simulink subsystem "Subsys_Conv_Ctrl_meas_Protection"  (R2022b)
settings: Solver=VariableStepAuto  StartTime=0.0  StopTime=10.0  RelTol=1e-3
model mask{prot_variant=1, f_n=50, meas_signals=0, v_n_dc=sqrt(6), v_dc_max=1.2*sqrt(6), v_ac_max=1.1, t_ac_max=0.1, v_ac_maxmax=1.25, t_ac_maxmax=0.1, v_ac_min=0.8, t_ac_min=3, v_ac_minmin=0.45, t_ac_minmin=0.3, f_ac_max=51.5, t_f_ac_max=0.1, f_ac_maxmax=52.5, t_f_ac_maxmax=10, f_ac_min=47.5, t_f_ac_min=0.1, i_ac_max=1.25, T_s=1e-4}
  mask prompts: prot_variant "Protection Variant (1 = hardware protection, 2 = tDMSquared warnings only, 3 = deactivated, 4 = VDE AR)"; f_n "Nominal frequency"; meas_signals "Measurement signals (0 = all signals (tDMSquared simulation), 1 = reduced (imperix hardware))"; v_n_dc "Nominal DC-link voltage [pu]"; v_dc_max "Maximum DC-link voltage [pu]"; v_ac_max "Maximum AC voltage amplitude [pu]"; t_ac_max "Maximum AC voltage amplitude timing"; v_ac_maxmax "Upper Maximum AC voltage amplitude [pu]"; t_ac_maxmax "Upper Maximum AC voltage amplitude timing"; v_ac_min "Upper Minimum AC voltage amplitude [pu]"; t_ac_min "Upper Minimum AC voltage amplitude timing"; v_ac_minmin "Lower Minimum AC voltage amplitude [pu]"; t_ac_minmin "Lower Minimum AC voltage amplitude timing"; f_ac_max "Maximum AC voltage frequency [Hz]"; t_f_ac_max "Maximum AC voltage frequency timing"; f_ac_maxmax "Upper Maximum AC voltage frequency [Hz]"; t_f_ac_maxmax "Upper Maximum AC voltage frequency timing"; f_ac_min "Minimum AC voltage frequency [Hz]"; t_f_ac_min "Minimum AC voltage frequencytiming"; i_ac_max "Maximum AC current amplitude [pu]"; T_s "Sample Time [s]"
undefined symbols (not defined in the file): DiscIntNeverNeededParam
libraries: simulink x63, spsRMSLib x1
settings Model: DefaultTestHarness=Subsys_Conv_Ctrl_meas_Protection_Harness1  Creator=winkens  LastModifiedBy=m.stroot
settings SolverCC: AlgebraicLoopSolver=TrustRegion
settings DebuggingCC: UnconnectedInputMsg=warning  UnconnectedOutputMsg=warning  UnconnectedLineMsg=warning  SFMachineParentedDataDiag=warning
settings ModelReferenceCC: EnableRefExpFcnMdlSchedulingChecks=on
settings RTWCC: DLArmComputeVersion=19.05

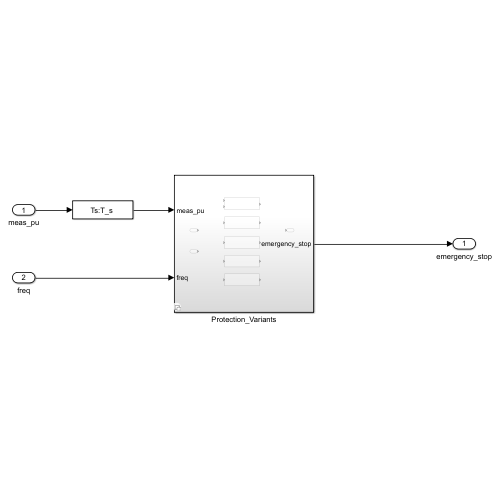
[thumbnail: Simulink's stored preview of the top-level diagram]
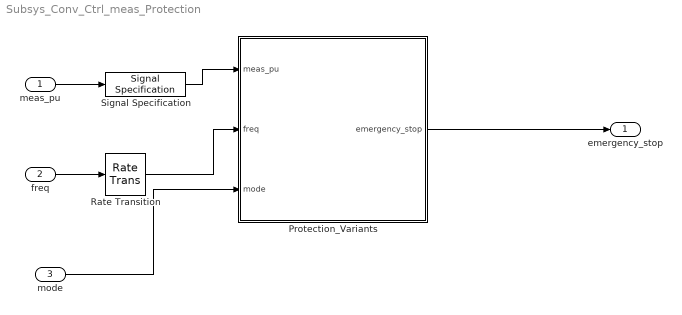
== system Subsys_Conv_Ctrl_meas_Protection ==
  meas_pu : Inport
  freq : Inport  Port=2
  mode : Inport  Port=3
  Protection_Variants : Subsystem  Variant=on
  Rate Transition : RateTransition  OutPortSampleTime=T_s
  Signal Specification : SignalSpecification  SampleTime=T_s
  emergency_stop : Outport  OutDataTypeStr=boolean
  wires:
  mode/1 -> Protection_Variants/3(mode)
  freq/1 -> Rate Transition/1
  Signal Specification/1 -> Protection_Variants/1(meas_pu)
  meas_pu/1 -> Signal Specification/1
  Protection_Variants/1(emergency_stop) -> emergency_stop/1
  Rate Transition/1 -> Protection_Variants/2(freq)

== system Subsys_Conv_Ctrl_meas_Protection/Protection_Variants ==
  meas_pu : Inport
  freq : Inport  Port=2
  mode : Inport  Port=3
  Hardware_Protection : Subsystem  VariantControl=(prot_variant == 1) && (meas_signals == 0)
  Hardware_Protection_imperix : Subsystem  VariantControl=(prot_variant == 1) && (meas_signals == 1)
  No_Protection : Subsystem  VariantControl=prot_variant == 3
  VDE_AR : Subsystem  VariantControl=(prot_variant == 4)
  tDMSquared_Warnings : Subsystem  VariantControl=prot_variant == 2
  emergency_stop : Outport

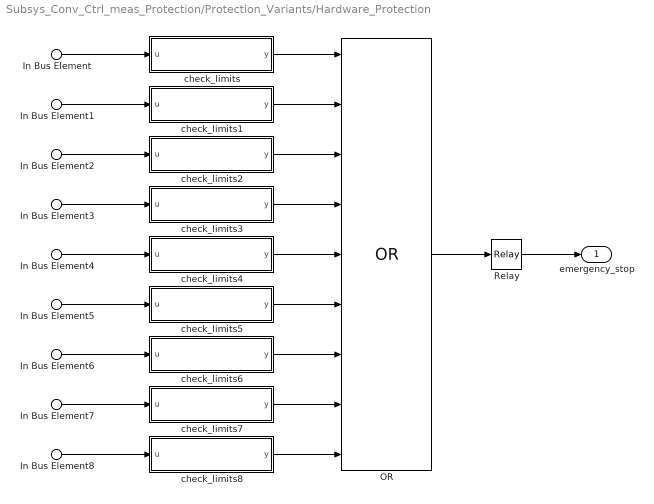
== system Subsys_Conv_Ctrl_meas_Protection/Protection_Variants/Hardware_Protection ==
  In Bus Element : Inport  PortName=meas_pu  Element=v_dc
  In Bus Element1 : Inport  PortName=meas_pu  Element=v_dc_up
  In Bus Element2 : Inport  PortName=meas_pu  Element=v_dc_low
  In Bus Element3 : Inport  PortName=meas_pu  Element=v_cap_abc
  In Bus Element4 : Inport  PortName=meas_pu  Element=v_breaker_abc
  In Bus Element5 : Inport  PortName=meas_pu  Element=v_grid_abc
  In Bus Element6 : Inport  PortName=meas_pu  Element=i_conv_abc
  In Bus Element7 : Inport  PortName=meas_pu  Element=i_filter_grid_abc
  In Bus Element8 : Inport  PortName=meas_pu  Element=i_grid_abc
  OR : Logic  Operator=OR  Inputs=9  AllPortsSameDT=off  OutDataTypeStr='double'
  Relay : Relay  OnSwitchValue=0.5  OffSwitchValue=-0.5  OutDataTypeStr=boolean
  check_limits : Subsystem
  check_limits1 : Subsystem
  check_limits2 : Subsystem
  check_limits3 : Subsystem
  check_limits4 : Subsystem
  check_limits5 : Subsystem
  check_limits6 : Subsystem
  check_limits7 : Subsystem
  check_limits8 : Subsystem
  emergency_stop : Outport
  wires:
  Relay/1 -> emergency_stop/1
  OR/1 -> Relay/1
  check_limits8/1(y) -> OR/9
  check_limits7/1(y) -> OR/8
  check_limits6/1(y) -> OR/7
  check_limits5/1(y) -> OR/6
  check_limits4/1(y) -> OR/5
  check_limits3/1(y) -> OR/4
  check_limits2/1(y) -> OR/3
  check_limits1/1(y) -> OR/2
  check_limits/1(y) -> OR/1
  In Bus Element8/1 -> check_limits8/1(u)
  In Bus Element7/1 -> check_limits7/1(u)
  In Bus Element6/1 -> check_limits6/1(u)
  In Bus Element4/1 -> check_limits4/1(u)
  In Bus Element5/1 -> check_limits5/1(u)
  In Bus Element3/1 -> check_limits3/1(u)
  In Bus Element2/1 -> check_limits2/1(u)
  In Bus Element1/1 -> check_limits1/1(u)
  In Bus Element/1 -> check_limits/1(u)

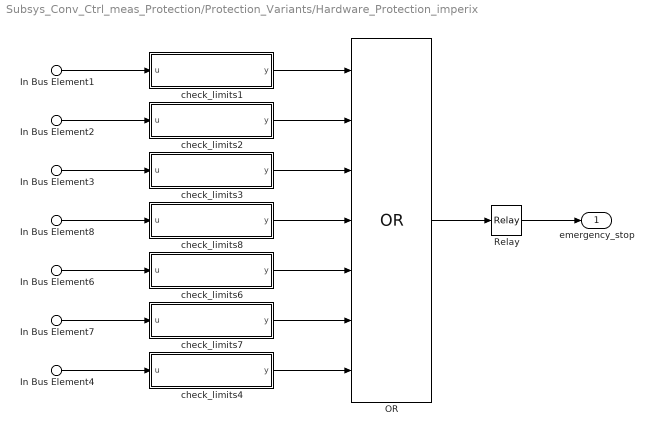
== system Subsys_Conv_Ctrl_meas_Protection/Protection_Variants/Hardware_Protection_imperix ==
  In Bus Element1 : Inport  PortName=meas_pu  Element=v_dc_up
  In Bus Element2 : Inport  PortName=meas_pu  Element=v_dc_low
  In Bus Element3 : Inport  PortName=meas_pu  Element=v_cap_ab-bc-ca
  In Bus Element6 : Inport  PortName=meas_pu  Element=i_conv2_abc
  In Bus Element7 : Inport  PortName=meas_pu  Element=i_filter_grid_abc
  In Bus Element8 : Inport  PortName=meas_pu  Element=i_conv1_abc
  In Bus Element4 : Inport  PortName=meas_pu  Element=i_filter_grid_n
  OR : Logic  Operator=OR  Inputs=7  AllPortsSameDT=off  OutDataTypeStr='double'
  Relay : Relay  OnSwitchValue=0.5  OffSwitchValue=-0.5  OutDataTypeStr=boolean
  check_limits1 : Subsystem
  check_limits2 : Subsystem
  check_limits3 : Subsystem
  check_limits4 : Subsystem
  check_limits6 : Subsystem
  check_limits7 : Subsystem
  check_limits8 : Subsystem
  emergency_stop : Outport
  wires:
  In Bus Element4/1 -> check_limits4/1(u)
  check_limits4/1(y) -> OR/7
  Relay/1 -> emergency_stop/1
  OR/1 -> Relay/1
  check_limits8/1(y) -> OR/4
  check_limits7/1(y) -> OR/6
  check_limits6/1(y) -> OR/5
  check_limits3/1(y) -> OR/3
  check_limits2/1(y) -> OR/2
  check_limits1/1(y) -> OR/1
  In Bus Element8/1 -> check_limits8/1(u)
  In Bus Element7/1 -> check_limits7/1(u)
  In Bus Element6/1 -> check_limits6/1(u)
  In Bus Element3/1 -> check_limits3/1(u)
  In Bus Element2/1 -> check_limits2/1(u)
  In Bus Element1/1 -> check_limits1/1(u)

== system Subsys_Conv_Ctrl_meas_Protection/Protection_Variants/No_Protection ==
  meas_pu : Inport
  Ground : Ground
  Terminator : Terminator
  emergency_stop : Outport
  wires:
  Ground/1 -> emergency_stop/1
  meas_pu/1 -> Terminator/1

== system Subsys_Conv_Ctrl_meas_Protection/Protection_Variants/VDE_AR ==
  In Bus Element1 : Inport  PortName=meas_pu  Element=v_breaker_abc
  freq : Inport  Port=2
  mode : Inport  Port=3
  Compare To Constant : simulink/Logic and Bit Operations/Compare To Constant  relop=>  const=1  OutDataTypeStr=boolean
  Subsystem : Subsystem
  emergency_stop : Outport
  wires:
  In Bus Element1/1 -> Subsystem/1(In1)
  freq/1 -> Subsystem/2(freq)
  Subsystem/1(emergency_stop) -> emergency_stop/1
  mode/1 -> Compare To Constant/1
  Compare To Constant/1 -> Subsystem/Enable

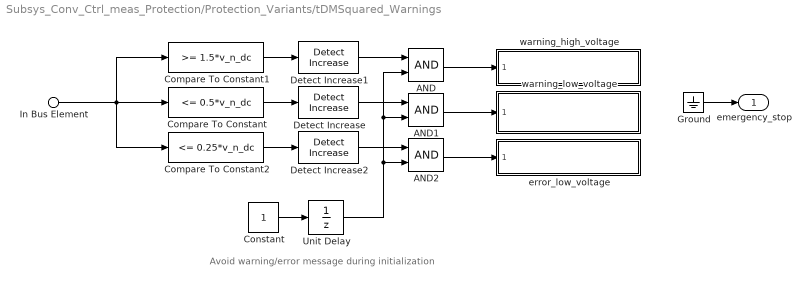
== system Subsys_Conv_Ctrl_meas_Protection/Protection_Variants/tDMSquared_Warnings ==
  note: Avoid warning/error message during initialization
  In Bus Element : Inport  PortName=meas_pu  Element=v_dc
  AND : Logic  AllPortsSameDT=off  OutDataTypeStr=boolean
  AND1 : Logic  AllPortsSameDT=off  OutDataTypeStr=boolean
  AND2 : Logic  AllPortsSameDT=off  OutDataTypeStr=boolean
  Compare To Constant : simulink/Logic and Bit Operations/Compare To Constant  relop=<=  const=0.5*v_n_dc  OutDataTypeStr=boolean
  Compare To Constant1 : simulink/Logic and Bit Operations/Compare To Constant  relop=>=  const=1.5*v_n_dc  OutDataTypeStr=boolean
  Compare To Constant2 : simulink/Logic and Bit Operations/Compare To Constant  relop=<=  const=0.25*v_n_dc  OutDataTypeStr=boolean
  Constant : Constant  OutDataTypeStr=boolean
  Detect Increase : simulink/Logic and Bit Operations/Detect Increase  vinit=0.0  OutDataTypeStr=boolean
  Detect Increase1 : simulink/Logic and Bit Operations/Detect Increase  vinit=0.0  OutDataTypeStr=boolean
  Detect Increase2 : simulink/Logic and Bit Operations/Detect Increase  vinit=0.0  OutDataTypeStr=boolean
  Ground : Ground
  Unit Delay : UnitDelay  SampleTime=T_s  HasFrameUpgradeWarning=on
  error_low_voltage : Subsystem  ReferencedSubsystem=tDMSquared_Error  messageText='DC-Link Voltage dropped below 25% of its nominal value. The simulation is terminated.'  T_s=T_s  stopSim=on
  warning_high_voltage : Subsystem  ReferencedSubsystem=tDMSquared_Warning  messageText='DC-Link Voltage increased to 150% of its nominal value. The results of the following timesteps need to be revisited.'  T_s=T_s
  warning_low_voltage : Subsystem  ReferencedSubsystem=tDMSquared_Warning  messageText='DC-Link Voltage dropped below 50% of its nominal value. The results of the following timesteps need to be revisited.'  T_s=T_s
  emergency_stop : Outport
  wires:
  Unit Delay/1 -> AND1/2, AND/2, AND2/2
  AND2/1 -> error_low_voltage/1
  AND1/1 -> warning_low_voltage/1
  AND/1 -> warning_high_voltage/1
  Constant/1 -> Unit Delay/1
  Compare To Constant/1 -> Detect Increase/1
  Compare To Constant2/1 -> Detect Increase2/1
  Detect Increase/1 -> AND1/1
  Compare To Constant1/1 -> Detect Increase1/1
  In Bus Element/1 -> Compare To Constant/1, Compare To Constant1/1, Compare To Constant2/1
  Detect Increase1/1 -> AND/1
  Detect Increase2/1 -> AND2/1
  Ground/1 -> emergency_stop/1

== system Subsys_Conv_Ctrl_meas_Protection/Protection_Variants/Hardware_Protection/check_limits ==
  u : Inport
  Compare To Constant1 : simulink/Logic and Bit Operations/Compare To Constant  relop=>=  const=v_dc_max  OutDataTypeStr=boolean
  y : Outport
  wires:
  u/1 -> Compare To Constant1/1
  Compare To Constant1/1 -> y/1

== system Subsys_Conv_Ctrl_meas_Protection/Protection_Variants/Hardware_Protection/check_limits1 ==
  u : Inport
  Compare To Constant1 : simulink/Logic and Bit Operations/Compare To Constant  relop=>=  const=0.5*v_dc_max  OutDataTypeStr=boolean
  y : Outport
  wires:
  u/1 -> Compare To Constant1/1
  Compare To Constant1/1 -> y/1

== system Subsys_Conv_Ctrl_meas_Protection/Protection_Variants/Hardware_Protection/check_limits2 ==
  u : Inport
  Compare To Constant1 : simulink/Logic and Bit Operations/Compare To Constant  relop=>=  const=0.5*v_dc_max  OutDataTypeStr=boolean
  y : Outport
  wires:
  u/1 -> Compare To Constant1/1
  Compare To Constant1/1 -> y/1

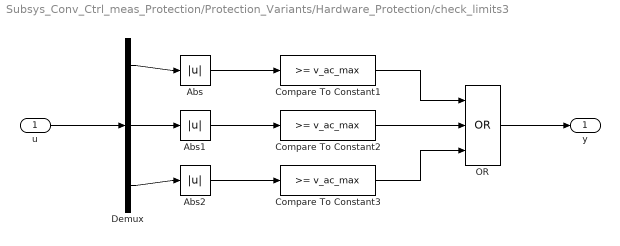
== system Subsys_Conv_Ctrl_meas_Protection/Protection_Variants/Hardware_Protection/check_limits3 ==
  u : Inport
  Abs : Abs  SaturateOnIntegerOverflow=off
  Abs1 : Abs  SaturateOnIntegerOverflow=off
  Abs2 : Abs  SaturateOnIntegerOverflow=off
  Compare To Constant1 : simulink/Logic and Bit Operations/Compare To Constant  relop=>=  const=v_ac_max  OutDataTypeStr=boolean
  Compare To Constant2 : simulink/Logic and Bit Operations/Compare To Constant  relop=>=  const=v_ac_max  OutDataTypeStr=boolean
  Compare To Constant3 : simulink/Logic and Bit Operations/Compare To Constant  relop=>=  const=v_ac_max  OutDataTypeStr=boolean
  Demux : Demux  Outputs=3
  OR : Logic  Operator=OR  Inputs=3  AllPortsSameDT=off  OutDataTypeStr=boolean
  y : Outport
  wires:
  OR/1 -> y/1
  Compare To Constant3/1 -> OR/3
  Compare To Constant1/1 -> OR/1
  Compare To Constant2/1 -> OR/2
  Abs2/1 -> Compare To Constant3/1
  Abs1/1 -> Compare To Constant2/1
  Abs/1 -> Compare To Constant1/1
  Demux/3 -> Abs2/1
  Demux/2 -> Abs1/1
  Demux/1 -> Abs/1
  u/1 -> Demux/1

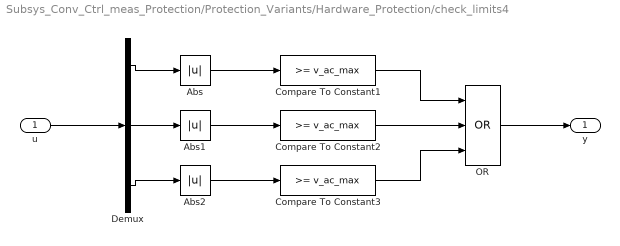
== system Subsys_Conv_Ctrl_meas_Protection/Protection_Variants/Hardware_Protection/check_limits4 ==
  u : Inport
  Abs : Abs  SaturateOnIntegerOverflow=off
  Abs1 : Abs  SaturateOnIntegerOverflow=off
  Abs2 : Abs  SaturateOnIntegerOverflow=off
  Compare To Constant1 : simulink/Logic and Bit Operations/Compare To Constant  relop=>=  const=v_ac_max  OutDataTypeStr=boolean
  Compare To Constant2 : simulink/Logic and Bit Operations/Compare To Constant  relop=>=  const=v_ac_max  OutDataTypeStr=boolean
  Compare To Constant3 : simulink/Logic and Bit Operations/Compare To Constant  relop=>=  const=v_ac_max  OutDataTypeStr=boolean
  Demux : Demux  Outputs=3
  OR : Logic  Operator=OR  Inputs=3  AllPortsSameDT=off  OutDataTypeStr=boolean
  y : Outport
  wires:
  OR/1 -> y/1
  Compare To Constant3/1 -> OR/3
  Compare To Constant1/1 -> OR/1
  Compare To Constant2/1 -> OR/2
  Abs2/1 -> Compare To Constant3/1
  Abs1/1 -> Compare To Constant2/1
  Abs/1 -> Compare To Constant1/1
  Demux/3 -> Abs2/1
  Demux/2 -> Abs1/1
  Demux/1 -> Abs/1
  u/1 -> Demux/1

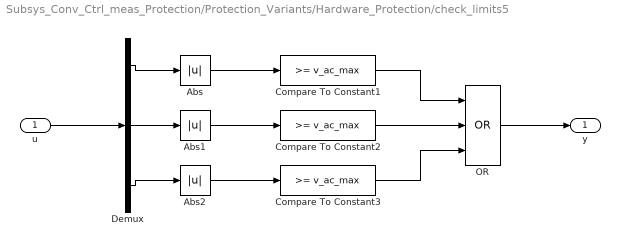
== system Subsys_Conv_Ctrl_meas_Protection/Protection_Variants/Hardware_Protection/check_limits5 ==
  u : Inport
  Abs : Abs  SaturateOnIntegerOverflow=off
  Abs1 : Abs  SaturateOnIntegerOverflow=off
  Abs2 : Abs  SaturateOnIntegerOverflow=off
  Compare To Constant1 : simulink/Logic and Bit Operations/Compare To Constant  relop=>=  const=v_ac_max  OutDataTypeStr=boolean
  Compare To Constant2 : simulink/Logic and Bit Operations/Compare To Constant  relop=>=  const=v_ac_max  OutDataTypeStr=boolean
  Compare To Constant3 : simulink/Logic and Bit Operations/Compare To Constant  relop=>=  const=v_ac_max  OutDataTypeStr=boolean
  Demux : Demux  Outputs=3
  OR : Logic  Operator=OR  Inputs=3  AllPortsSameDT=off  OutDataTypeStr=boolean
  y : Outport
  wires:
  OR/1 -> y/1
  Compare To Constant3/1 -> OR/3
  Compare To Constant1/1 -> OR/1
  Compare To Constant2/1 -> OR/2
  Abs2/1 -> Compare To Constant3/1
  Abs1/1 -> Compare To Constant2/1
  Abs/1 -> Compare To Constant1/1
  Demux/3 -> Abs2/1
  Demux/2 -> Abs1/1
  Demux/1 -> Abs/1
  u/1 -> Demux/1

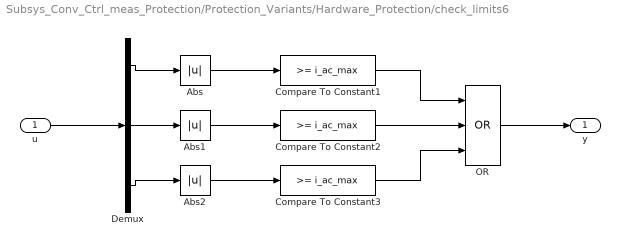
== system Subsys_Conv_Ctrl_meas_Protection/Protection_Variants/Hardware_Protection/check_limits6 ==
  u : Inport
  Abs : Abs  SaturateOnIntegerOverflow=off
  Abs1 : Abs  SaturateOnIntegerOverflow=off
  Abs2 : Abs  SaturateOnIntegerOverflow=off
  Compare To Constant1 : simulink/Logic and Bit Operations/Compare To Constant  relop=>=  const=i_ac_max  OutDataTypeStr=boolean
  Compare To Constant2 : simulink/Logic and Bit Operations/Compare To Constant  relop=>=  const=i_ac_max  OutDataTypeStr=boolean
  Compare To Constant3 : simulink/Logic and Bit Operations/Compare To Constant  relop=>=  const=i_ac_max  OutDataTypeStr=boolean
  Demux : Demux  Outputs=3
  OR : Logic  Operator=OR  Inputs=3  AllPortsSameDT=off  OutDataTypeStr=boolean
  y : Outport
  wires:
  OR/1 -> y/1
  Compare To Constant3/1 -> OR/3
  Compare To Constant1/1 -> OR/1
  Compare To Constant2/1 -> OR/2
  Abs2/1 -> Compare To Constant3/1
  Abs1/1 -> Compare To Constant2/1
  Abs/1 -> Compare To Constant1/1
  Demux/3 -> Abs2/1
  Demux/2 -> Abs1/1
  Demux/1 -> Abs/1
  u/1 -> Demux/1

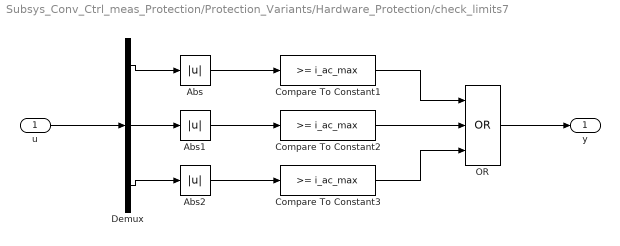
== system Subsys_Conv_Ctrl_meas_Protection/Protection_Variants/Hardware_Protection/check_limits7 ==
  u : Inport
  Abs : Abs  SaturateOnIntegerOverflow=off
  Abs1 : Abs  SaturateOnIntegerOverflow=off
  Abs2 : Abs  SaturateOnIntegerOverflow=off
  Compare To Constant1 : simulink/Logic and Bit Operations/Compare To Constant  relop=>=  const=i_ac_max  OutDataTypeStr=boolean
  Compare To Constant2 : simulink/Logic and Bit Operations/Compare To Constant  relop=>=  const=i_ac_max  OutDataTypeStr=boolean
  Compare To Constant3 : simulink/Logic and Bit Operations/Compare To Constant  relop=>=  const=i_ac_max  OutDataTypeStr=boolean
  Demux : Demux  Outputs=3
  OR : Logic  Operator=OR  Inputs=3  AllPortsSameDT=off  OutDataTypeStr=boolean
  y : Outport
  wires:
  OR/1 -> y/1
  Compare To Constant3/1 -> OR/3
  Compare To Constant1/1 -> OR/1
  Compare To Constant2/1 -> OR/2
  Abs2/1 -> Compare To Constant3/1
  Abs1/1 -> Compare To Constant2/1
  Abs/1 -> Compare To Constant1/1
  Demux/3 -> Abs2/1
  Demux/2 -> Abs1/1
  Demux/1 -> Abs/1
  u/1 -> Demux/1

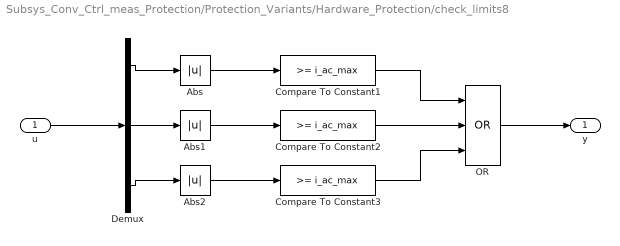
== system Subsys_Conv_Ctrl_meas_Protection/Protection_Variants/Hardware_Protection/check_limits8 ==
  u : Inport
  Abs : Abs  SaturateOnIntegerOverflow=off
  Abs1 : Abs  SaturateOnIntegerOverflow=off
  Abs2 : Abs  SaturateOnIntegerOverflow=off
  Compare To Constant1 : simulink/Logic and Bit Operations/Compare To Constant  relop=>=  const=i_ac_max  OutDataTypeStr=boolean
  Compare To Constant2 : simulink/Logic and Bit Operations/Compare To Constant  relop=>=  const=i_ac_max  OutDataTypeStr=boolean
  Compare To Constant3 : simulink/Logic and Bit Operations/Compare To Constant  relop=>=  const=i_ac_max  OutDataTypeStr=boolean
  Demux : Demux  Outputs=3
  OR : Logic  Operator=OR  Inputs=3  AllPortsSameDT=off  OutDataTypeStr=boolean
  y : Outport
  wires:
  OR/1 -> y/1
  Compare To Constant3/1 -> OR/3
  Compare To Constant1/1 -> OR/1
  Compare To Constant2/1 -> OR/2
  Abs2/1 -> Compare To Constant3/1
  Abs1/1 -> Compare To Constant2/1
  Abs/1 -> Compare To Constant1/1
  Demux/3 -> Abs2/1
  Demux/2 -> Abs1/1
  Demux/1 -> Abs/1
  u/1 -> Demux/1

== system Subsys_Conv_Ctrl_meas_Protection/Protection_Variants/Hardware_Protection_imperix/check_limits1 ==
  u : Inport
  Compare To Constant1 : simulink/Logic and Bit Operations/Compare To Constant  relop=>=  const=0.5*v_dc_max  OutDataTypeStr=boolean
  y : Outport
  wires:
  u/1 -> Compare To Constant1/1
  Compare To Constant1/1 -> y/1

== system Subsys_Conv_Ctrl_meas_Protection/Protection_Variants/Hardware_Protection_imperix/check_limits2 ==
  u : Inport
  Compare To Constant1 : simulink/Logic and Bit Operations/Compare To Constant  relop=>=  const=0.5*v_dc_max  OutDataTypeStr=boolean
  y : Outport
  wires:
  u/1 -> Compare To Constant1/1
  Compare To Constant1/1 -> y/1

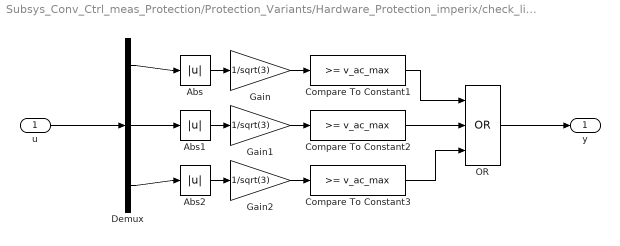
== system Subsys_Conv_Ctrl_meas_Protection/Protection_Variants/Hardware_Protection_imperix/check_limits3 ==
  u : Inport
  Abs : Abs  SaturateOnIntegerOverflow=off
  Abs1 : Abs  SaturateOnIntegerOverflow=off
  Abs2 : Abs  SaturateOnIntegerOverflow=off
  Compare To Constant1 : simulink/Logic and Bit Operations/Compare To Constant  relop=>=  const=v_ac_max  OutDataTypeStr=boolean
  Compare To Constant2 : simulink/Logic and Bit Operations/Compare To Constant  relop=>=  const=v_ac_max  OutDataTypeStr=boolean
  Compare To Constant3 : simulink/Logic and Bit Operations/Compare To Constant  relop=>=  const=v_ac_max  OutDataTypeStr=boolean
  Demux : Demux  Outputs=3
  Gain : Gain  Gain=1/sqrt(3)
  Gain1 : Gain  Gain=1/sqrt(3)
  Gain2 : Gain  Gain=1/sqrt(3)
  OR : Logic  Operator=OR  Inputs=3  AllPortsSameDT=off  OutDataTypeStr=boolean
  y : Outport
  wires:
  OR/1 -> y/1
  Compare To Constant3/1 -> OR/3
  Compare To Constant1/1 -> OR/1
  Compare To Constant2/1 -> OR/2
  Abs2/1 -> Gain2/1
  Abs1/1 -> Gain1/1
  Abs/1 -> Gain/1
  Demux/3 -> Abs2/1
  Demux/2 -> Abs1/1
  Demux/1 -> Abs/1
  u/1 -> Demux/1
  Gain/1 -> Compare To Constant1/1
  Gain1/1 -> Compare To Constant2/1
  Gain2/1 -> Compare To Constant3/1

== system Subsys_Conv_Ctrl_meas_Protection/Protection_Variants/Hardware_Protection_imperix/check_limits4 ==
  u : Inport
  Abs : Abs  SaturateOnIntegerOverflow=off
  Compare To Constant1 : simulink/Logic and Bit Operations/Compare To Constant  relop=>=  const=i_ac_max  OutDataTypeStr=boolean
  y : Outport
  wires:
  Compare To Constant1/1 -> y/1
  Abs/1 -> Compare To Constant1/1
  u/1 -> Abs/1

== system Subsys_Conv_Ctrl_meas_Protection/Protection_Variants/Hardware_Protection_imperix/check_limits6 ==
  u : Inport
  Abs : Abs  SaturateOnIntegerOverflow=off
  Abs1 : Abs  SaturateOnIntegerOverflow=off
  Abs2 : Abs  SaturateOnIntegerOverflow=off
  Compare To Constant1 : simulink/Logic and Bit Operations/Compare To Constant  relop=>=  const=i_ac_max  OutDataTypeStr=boolean
  Compare To Constant2 : simulink/Logic and Bit Operations/Compare To Constant  relop=>=  const=i_ac_max  OutDataTypeStr=boolean
  Compare To Constant3 : simulink/Logic and Bit Operations/Compare To Constant  relop=>=  const=i_ac_max  OutDataTypeStr=boolean
  Demux : Demux  Outputs=3
  OR : Logic  Operator=OR  Inputs=3  AllPortsSameDT=off  OutDataTypeStr=boolean
  y : Outport
  wires:
  OR/1 -> y/1
  Compare To Constant3/1 -> OR/3
  Compare To Constant1/1 -> OR/1
  Compare To Constant2/1 -> OR/2
  Abs2/1 -> Compare To Constant3/1
  Abs1/1 -> Compare To Constant2/1
  Abs/1 -> Compare To Constant1/1
  Demux/3 -> Abs2/1
  Demux/2 -> Abs1/1
  Demux/1 -> Abs/1
  u/1 -> Demux/1

== system Subsys_Conv_Ctrl_meas_Protection/Protection_Variants/Hardware_Protection_imperix/check_limits7 ==
  u : Inport
  Abs : Abs  SaturateOnIntegerOverflow=off
  Abs1 : Abs  SaturateOnIntegerOverflow=off
  Abs2 : Abs  SaturateOnIntegerOverflow=off
  Compare To Constant1 : simulink/Logic and Bit Operations/Compare To Constant  relop=>=  const=i_ac_max  OutDataTypeStr=boolean
  Compare To Constant2 : simulink/Logic and Bit Operations/Compare To Constant  relop=>=  const=i_ac_max  OutDataTypeStr=boolean
  Compare To Constant3 : simulink/Logic and Bit Operations/Compare To Constant  relop=>=  const=i_ac_max  OutDataTypeStr=boolean
  Demux : Demux  Outputs=3
  OR : Logic  Operator=OR  Inputs=3  AllPortsSameDT=off  OutDataTypeStr=boolean
  y : Outport
  wires:
  OR/1 -> y/1
  Compare To Constant3/1 -> OR/3
  Compare To Constant1/1 -> OR/1
  Compare To Constant2/1 -> OR/2
  Abs2/1 -> Compare To Constant3/1
  Abs1/1 -> Compare To Constant2/1
  Abs/1 -> Compare To Constant1/1
  Demux/3 -> Abs2/1
  Demux/2 -> Abs1/1
  Demux/1 -> Abs/1
  u/1 -> Demux/1

== system Subsys_Conv_Ctrl_meas_Protection/Protection_Variants/Hardware_Protection_imperix/check_limits8 ==
  u : Inport
  Abs : Abs  SaturateOnIntegerOverflow=off
  Abs1 : Abs  SaturateOnIntegerOverflow=off
  Abs2 : Abs  SaturateOnIntegerOverflow=off
  Compare To Constant1 : simulink/Logic and Bit Operations/Compare To Constant  relop=>=  const=i_ac_max  OutDataTypeStr=boolean
  Compare To Constant2 : simulink/Logic and Bit Operations/Compare To Constant  relop=>=  const=i_ac_max  OutDataTypeStr=boolean
  Compare To Constant3 : simulink/Logic and Bit Operations/Compare To Constant  relop=>=  const=i_ac_max  OutDataTypeStr=boolean
  Demux : Demux  Outputs=3
  OR : Logic  Operator=OR  Inputs=3  AllPortsSameDT=off  OutDataTypeStr=boolean
  y : Outport
  wires:
  OR/1 -> y/1
  Compare To Constant3/1 -> OR/3
  Compare To Constant1/1 -> OR/1
  Compare To Constant2/1 -> OR/2
  Abs2/1 -> Compare To Constant3/1
  Abs1/1 -> Compare To Constant2/1
  Abs/1 -> Compare To Constant1/1
  Demux/3 -> Abs2/1
  Demux/2 -> Abs1/1
  Demux/1 -> Abs/1
  u/1 -> Demux/1

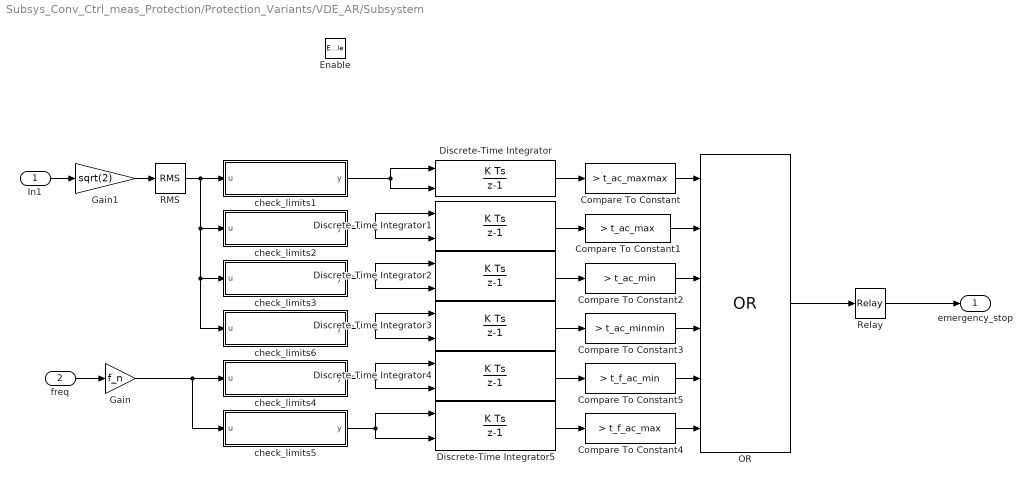
== system Subsys_Conv_Ctrl_meas_Protection/Protection_Variants/VDE_AR/Subsystem ==
  In1 : Inport
  freq : Inport  Port=2
  Enable : EnablePort
  Compare To Constant : simulink/Logic and Bit Operations/Compare To Constant  relop=>  const=t_ac_maxmax  OutDataTypeStr=boolean
  Compare To Constant1 : simulink/Logic and Bit Operations/Compare To Constant  relop=>  const=t_ac_max  OutDataTypeStr=boolean
  Compare To Constant2 : simulink/Logic and Bit Operations/Compare To Constant  relop=>  const=t_ac_min  OutDataTypeStr=boolean
  Compare To Constant3 : simulink/Logic and Bit Operations/Compare To Constant  relop=>  const=t_ac_minmin  OutDataTypeStr=boolean
  Compare To Constant4 : simulink/Logic and Bit Operations/Compare To Constant  relop=>  const=t_f_ac_max  OutDataTypeStr=boolean
  Compare To Constant5 : simulink/Logic and Bit Operations/Compare To Constant  relop=>  const=t_f_ac_min  OutDataTypeStr=boolean
  Discrete-Time Integrator : DiscreteIntegrator  ExternalReset=falling  SampleTime=-1  OutDataTypeStr=Inherit: Inherit via back propagation  LimitOutput=on  UpperSaturationLimit=10  LowerSaturationLimit=0  ICPrevOutput=DiscIntNeverNeededParam  ICPrevScaledInput=DiscIntNeverNeededParam
  Discrete-Time Integrator{1..5} (5 alike) : DiscreteIntegrator  ExternalReset=falling  SampleTime=-1  OutDataTypeStr=Inherit: Inherit via back propagation  LimitOutput=on  UpperSaturationLimit=10  LowerSaturationLimit=0  IgnoreLimit=on  ICPrevOutput=DiscIntNeverNeededParam  ICPrevScaledInput=DiscIntNeverNeededParam
  Gain : Gain  Gain=f_n
  Gain1 : Gain  Gain=sqrt(2)
  OR : Logic  Operator=OR  Inputs=6  AllPortsSameDT=off  OutDataTypeStr='double'
  RMS : spsRMSLib/RMS  TrueRMS=on  Freq=50  RMSInit=1  Ts=T_s
  Relay : Relay  OnSwitchValue=0.5  OffSwitchValue=-0.5  OutDataTypeStr=boolean
  check_limits1 : Subsystem
  check_limits2 : Subsystem
  check_limits3 : Subsystem
  check_limits4 : Subsystem
  check_limits5 : Subsystem
  check_limits6 : Subsystem
  emergency_stop : Outport
  wires:
  check_limits5/1(y) -> Discrete-Time Integrator5/1, Discrete-Time Integrator5/2
  Compare To Constant5/1 -> OR/5
  Relay/1 -> emergency_stop/1
  check_limits1/1(y) -> Discrete-Time Integrator/2, Discrete-Time Integrator/1
  check_limits4/1(y) -> Discrete-Time Integrator4/1, Discrete-Time Integrator4/2
  RMS/1 -> check_limits1/1(u), check_limits6/1(u), check_limits3/1(u), check_limits2/1(u)
  In1/1 -> Gain1/1
  Gain1/1 -> RMS/1
  Discrete-Time Integrator2/1 -> Compare To Constant2/1
  Discrete-Time Integrator/1 -> Compare To Constant/1
  check_limits3/1(y) -> Discrete-Time Integrator2/1, Discrete-Time Integrator2/2
  freq/1 -> Gain/1
  Discrete-Time Integrator5/1 -> Compare To Constant4/1
  Gain/1 -> check_limits4/1(u), check_limits5/1(u)
  Compare To Constant4/1 -> OR/6
  Discrete-Time Integrator1/1 -> Compare To Constant1/1
  check_limits2/1(y) -> Discrete-Time Integrator1/1, Discrete-Time Integrator1/2
  Compare To Constant2/1 -> OR/3
  check_limits6/1(y) -> Discrete-Time Integrator3/1, Discrete-Time Integrator3/2
  Compare To Constant3/1 -> OR/4
  Compare To Constant1/1 -> OR/2
  Discrete-Time Integrator3/1 -> Compare To Constant3/1
  Discrete-Time Integrator4/1 -> Compare To Constant5/1
  OR/1 -> Relay/1
  Compare To Constant/1 -> OR/1

== system Subsys_Conv_Ctrl_meas_Protection/Protection_Variants/VDE_AR/Subsystem/check_limits1 ==
  u : Inport
  Compare To Constant1 : simulink/Logic and Bit Operations/Compare To Constant  relop=>=  const=v_ac_maxmax  OutDataTypeStr=boolean
  Compare To Constant2 : simulink/Logic and Bit Operations/Compare To Constant  relop=>=  const=v_ac_maxmax  OutDataTypeStr=boolean
  Compare To Constant3 : simulink/Logic and Bit Operations/Compare To Constant  relop=>=  const=v_ac_maxmax  OutDataTypeStr=boolean
  Demux : Demux  Outputs=3
  OR : Logic  Operator=OR  Inputs=3  AllPortsSameDT=off  OutDataTypeStr=boolean
  y : Outport
  wires:
  OR/1 -> y/1
  Compare To Constant3/1 -> OR/3
  Compare To Constant1/1 -> OR/1
  Compare To Constant2/1 -> OR/2
  Demux/3 -> Compare To Constant3/1
  Demux/2 -> Compare To Constant2/1
  Demux/1 -> Compare To Constant1/1
  u/1 -> Demux/1

== system Subsys_Conv_Ctrl_meas_Protection/Protection_Variants/VDE_AR/Subsystem/check_limits2 ==
  u : Inport
  Compare To Constant1 : simulink/Logic and Bit Operations/Compare To Constant  relop=>=  const=v_ac_max  OutDataTypeStr=boolean
  Compare To Constant2 : simulink/Logic and Bit Operations/Compare To Constant  relop=>=  const=v_ac_max  OutDataTypeStr=boolean
  Compare To Constant3 : simulink/Logic and Bit Operations/Compare To Constant  relop=>=  const=v_ac_max  OutDataTypeStr=boolean
  Demux : Demux  Outputs=3
  OR : Logic  Operator=OR  Inputs=3  AllPortsSameDT=off  OutDataTypeStr=boolean
  y : Outport
  wires:
  OR/1 -> y/1
  Compare To Constant3/1 -> OR/3
  Compare To Constant1/1 -> OR/1
  Compare To Constant2/1 -> OR/2
  Demux/3 -> Compare To Constant3/1
  Demux/2 -> Compare To Constant2/1
  Demux/1 -> Compare To Constant1/1
  u/1 -> Demux/1

== system Subsys_Conv_Ctrl_meas_Protection/Protection_Variants/VDE_AR/Subsystem/check_limits3 ==
  u : Inport
  Compare To Constant1 : simulink/Logic and Bit Operations/Compare To Constant  relop=<=  const=v_ac_min  OutDataTypeStr=boolean
  Compare To Constant2 : simulink/Logic and Bit Operations/Compare To Constant  relop=<=  const=v_ac_min  OutDataTypeStr=boolean
  Compare To Constant3 : simulink/Logic and Bit Operations/Compare To Constant  relop=<=  const=v_ac_min  OutDataTypeStr=boolean
  Demux : Demux  Outputs=3
  OR : Logic  Operator=OR  Inputs=3  AllPortsSameDT=off  OutDataTypeStr=boolean
  y : Outport
  wires:
  OR/1 -> y/1
  Compare To Constant3/1 -> OR/3
  Compare To Constant1/1 -> OR/1
  Compare To Constant2/1 -> OR/2
  Demux/3 -> Compare To Constant3/1
  Demux/2 -> Compare To Constant2/1
  Demux/1 -> Compare To Constant1/1
  u/1 -> Demux/1

== system Subsys_Conv_Ctrl_meas_Protection/Protection_Variants/VDE_AR/Subsystem/check_limits4 ==
  u : Inport
  Compare To Constant1 : simulink/Logic and Bit Operations/Compare To Constant  relop=<=  const=f_ac_min  OutDataTypeStr=boolean
  y : Outport
  wires:
  Compare To Constant1/1 -> y/1
  u/1 -> Compare To Constant1/1

== system Subsys_Conv_Ctrl_meas_Protection/Protection_Variants/VDE_AR/Subsystem/check_limits5 ==
  u : Inport
  Compare To Constant1 : simulink/Logic and Bit Operations/Compare To Constant  relop=>=  const=f_ac_max  OutDataTypeStr=boolean
  y : Outport
  wires:
  Compare To Constant1/1 -> y/1
  u/1 -> Compare To Constant1/1

== system Subsys_Conv_Ctrl_meas_Protection/Protection_Variants/VDE_AR/Subsystem/check_limits6 ==
  u : Inport
  Compare To Constant1 : simulink/Logic and Bit Operations/Compare To Constant  relop=<=  const=v_ac_minmin  OutDataTypeStr=boolean
  Compare To Constant2 : simulink/Logic and Bit Operations/Compare To Constant  relop=<=  const=v_ac_minmin  OutDataTypeStr=boolean
  Compare To Constant3 : simulink/Logic and Bit Operations/Compare To Constant  relop=<=  const=v_ac_minmin  OutDataTypeStr=boolean
  Demux : Demux  Outputs=3
  OR : Logic  Operator=OR  Inputs=3  AllPortsSameDT=off  OutDataTypeStr=boolean
  y : Outport
  wires:
  OR/1 -> y/1
  Compare To Constant3/1 -> OR/3
  Compare To Constant1/1 -> OR/1
  Compare To Constant2/1 -> OR/2
  Demux/3 -> Compare To Constant3/1
  Demux/2 -> Compare To Constant2/1
  Demux/1 -> Compare To Constant1/1
  u/1 -> Demux/1
